simulink model "Pierre_Controller_LPV"  (R2024b)
settings: Solver=ode1  StartTime=0.0  StopTime=inf  FixedStep=Ts  RelTol=1e-3
PostLoadFcn:
  | , if any(exist('dsrtsu_mdlpostloadfcn', 'file') ~= 0), dsrtsu_mdlpostloadfcn('Execute', bdroot); end,
InitFcn:
  | , if any(exist('rtifpga_mdlclblib', 'file') ~= 0), rtifpga_mdlclblib('Init', bdroot); end,
model workspace (MAT data in the model file):
  dmestimate = 1
values from neighbouring files (symbols this model uses):
  BUTTER = ss(A,B,C,D,Ts)    [build_model.m]
  K = opensave.K_final    [build_model.m]
  Px = 1    [build_model.m]
  Py = 1    [build_model.m]
  Pz = 1    [build_model.m]
  S_Sensor = 0.1134    [build_model.m]
  Sen_AX = 2.0176    [build_model.m]
  Sen_AY = 2.011    [build_model.m]
  Sen_AZ = 2.0066    [build_model.m]
  Sen_GX = 0.75481    [build_model.m]
  Sen_GY = 0.75728    [build_model.m]
  Sen_GZ = 0.74931    [build_model.m]
  Sweep_amp = 0.5    [build_model.m]
  Switch_excit = 4    [build_model.m]
  TMS_amp = 2    [build_model.m]
  TMS_freq1 = 80    [build_model.m]
  TMS_freq2 = 0    [build_model.m]
  TMS_freq3 = 0    [build_model.m]
  Ts = 1/Fs    (= 0.001)    [build_model.m]
  V_sat = 2/10    (= 0.2)    [build_model.m]
  V_sat_TMS = 5    [build_model.m]
undefined symbols (not defined in the file or in its folder): dmhat, Gnomden, Gnomnum, R, S
libraries: dspfdesign x15, rti1202lib_adc_class1 x10, rti1202lib_dac_class1 x7, rti1202lib_adc_class2 x6, dspxfrm3 x3, cstblocks x1, simulink x1
(part 3 of 3)

== system Pierre_Controller_LPV/RTI Data ==
  RTI Data Store : Subsystem  Tag="struct('private',struct('version',struct('dsVer',uint32(2),'dsVerCreation',uint32(2),'RTI',struct('ver','7.18','type','RTI1202')),'access',struct('type','Model','isPerm',1,'created',['16-Aug-2022 11:52:04'],'modified',['22-Feb-2023 15:24:02'],'location','')),'public',struct('main',struct('data',[]),'sub',struct('name',{{'Pierre_Controller_LTI'}},'data',{{struct('TH',struct('thTaskInfo',struct('taskType',{'TIMER','HWINT','TMRINT','SWINT','GLINT'},'tasksNumOf',{1,0,0,0,0},'srcIds',{{'TIMERA'},{},{},{},{}},'taskNames',{{['Timer Task 1']},{},{},{},{}})),'th_tc',struct('dataType','TASK','taskGroupId','','taskGroupList',{{}},'taskSchedulingPolicy','FCFS','taskType','TIMER','blkh',-1,'srcId','TIMERA','srcSgnName',['Timer A interrupt'],'srcCpuName','','taskName',['Timer Task 1  [0.001] s'],'taskNameDisplayExt','','smplTime',0.001,'smplTimeOffs',0,'hasFixedPriority',0,'priority',1,'hasFixedOvc',0,'ovcType',1,'ovcMax',1),'tc_th',struct('dataType','TASK','taskGroupId','','taskGroupList',{{}},'taskSchedulingPolicy','FCFS','taskType','TIMER','blkh',-1,'srcId','TIMERA','srcSgnName',['Timer A interrupt'],'srcCpuName','','taskName',['Timer Task 1  [0.001] s'],'taskNameDisplayExt','','smplTime',0.001,'smplTimeOffs',0,'hasFixedPriority',0,'priority',1,'hasFixedOvc',0,'ovcType',1,'ovcMax',1))}})))"  mask(RTI_DATA_STORE){}
      mask help:
      | RTI Data Store Block. This block is used by RTI to store internal model dependent data. Deleting this block will result in data loss.
      |
      | NEVER DELETE, COPY, OR MODIFY THIS BLOCK!
      mask Help:
      | RTI Data Store Block. This block is used by RTI to store internal model dependent data. Deleting this block will result in data loss.
      | 
      | NEVER DELETE, COPY, OR MODIFY THIS BLOCK!
      mask Display: text(0.5, 0.5, ' ', 'HorizontalAlignment', 'center');

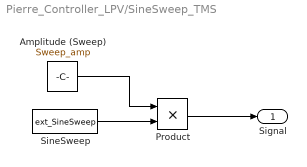
== system Pierre_Controller_LPV/SineSweep_TMS ==
  Amplitude (Sweep) : Constant  Value=Sweep_amp
  Product : Product
  SineSweep : FromWorkspace  VariableName=ext_SineSweep  SampleTime=Ts  Interpolate=off  OutputAfterFinalValue=Cyclic repetition
  Signal : Outport  VectorParamsAs1DForOutWhenUnconnected=off
  wires:
  Product/1 -> Signal/1
  SineSweep/1 -> Product/2
  Amplitude (Sweep)/1 -> Product/1

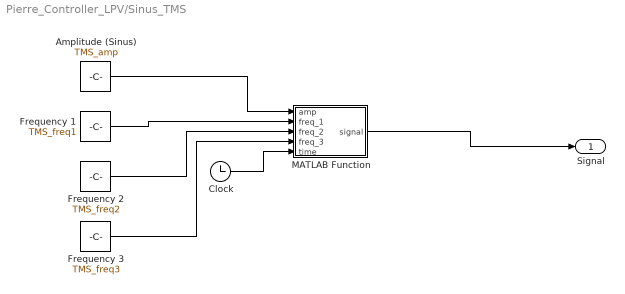
== system Pierre_Controller_LPV/Sinus_TMS ==
  Amplitude (Sinus) : Constant  Value=TMS_amp
  Clock : Clock
  Frequency 1 : Constant  Value=TMS_freq1
  Frequency 2 : Constant  Value=TMS_freq2
  Frequency 3 : Constant  Value=TMS_freq3
  MATLAB Function : MATLAB Function  TreatAsAtomicUnit=on
  Signal : Outport  VectorParamsAs1DForOutWhenUnconnected=off
  wires:
  Frequency 1/1 -> MATLAB Function/2(freq_1)
  Clock/1 -> MATLAB Function/5(time)
  Amplitude (Sinus)/1 -> MATLAB Function/1(amp)
  MATLAB Function/1(signal) -> Signal/1
  Frequency 2/1 -> MATLAB Function/3(freq_2)
  Frequency 3/1 -> MATLAB Function/4(freq_3)

== system Pierre_Controller_LPV/TMS_Command ==
  In1 : Inport
  GainDAC_Ch1 : Gain  Gain=1/10
  Command (V) : Outport  VectorParamsAs1DForOutWhenUnconnected=off
  wires:
  GainDAC_Ch1/1 -> Command (V)/1  "Command (V)"
  In1/1 -> GainDAC_Ch1/1

== system Pierre_Controller_LPV/ARCHIVE/Compensation filter ==
  Reference : Inport
  Compensation filter : cstblocks/LTI System  sys=Cz  IC=[]  PadeOrder=0
  Filtered Reference : Outport  VectorParamsAs1DForOutWhenUnconnected=off
  wires:
  Compensation filter/1 -> Filtered Reference/1
  Reference/1 -> Compensation filter/1

== system Pierre_Controller_LPV/ARCHIVE/SineSweep ==
  Amplitude (Sweep) : Constant
  Product : Product
  SineSweep : FromWorkspace  VariableName=ext_SineSweep  SampleTime=Ts  Interpolate=off  OutputAfterFinalValue=Cyclic repetition
  Signal : Outport  VectorParamsAs1DForOutWhenUnconnected=off
  wires:
  Amplitude (Sweep)/1 -> Product/1
  Product/1 -> Signal/1
  SineSweep/1 -> Product/2

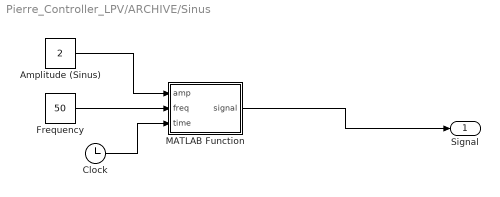
== system Pierre_Controller_LPV/ARCHIVE/Sinus ==
  Amplitude (Sinus) : Constant  Value=2
  Clock : Clock
  Frequency : Constant  Value=50
  MATLAB Function : MATLAB Function  TreatAsAtomicUnit=on
  Signal : Outport  VectorParamsAs1DForOutWhenUnconnected=off
  wires:
  Frequency/1 -> MATLAB Function/2(freq)
  Clock/1 -> MATLAB Function/3(time)
  Amplitude (Sinus)/1 -> MATLAB Function/1(amp)
  MATLAB Function/1(signal) -> Signal/1

== system Pierre_Controller_LPV/Current monitoring/Subsystem ==
  In1 : Inport
  V2A_PMA_monitoring : Gain  Gain=1/5
  PMA1_monitoring (A) : Outport  VectorParamsAs1DForOutWhenUnconnected=off
  wires:
  In1/1 -> V2A_PMA_monitoring/1
  V2A_PMA_monitoring/1 -> PMA1_monitoring (A)/1  "PMA_monitoring (A)"

== system Pierre_Controller_LPV/Current monitoring/Subsystem1 ==
  In1 : Inport
  V2A_PMA_monitoring : Gain  Gain=1/5
  PMA2_monitoring (A) : Outport  VectorParamsAs1DForOutWhenUnconnected=off
  wires:
  In1/1 -> V2A_PMA_monitoring/1
  V2A_PMA_monitoring/1 -> PMA2_monitoring (A)/1  "PMA_monitoring (A)"

== system Pierre_Controller_LPV/Current monitoring/Subsystem2 ==
  In1 : Inport
  V2A_PMA_monitoring : Gain  Gain=1/5
  PMA3_monitoring (A) : Outport  VectorParamsAs1DForOutWhenUnconnected=off
  wires:
  In1/1 -> V2A_PMA_monitoring/1
  V2A_PMA_monitoring/1 -> PMA3_monitoring (A)/1  "PMA_monitoring (A)"

== system Pierre_Controller_LPV/Current monitoring/Subsystem3 ==
  In1 : Inport
  V2A_PMA_monitoring : Gain  Gain=1/5
  PMA4_monitoring (A) : Outport  VectorParamsAs1DForOutWhenUnconnected=off
  wires:
  In1/1 -> V2A_PMA_monitoring/1
  V2A_PMA_monitoring/1 -> PMA4_monitoring (A)/1  "PMA_monitoring (A)"

== system Pierre_Controller_LPV/Current monitoring/Subsystem4 ==
  In1 : Inport
  V2A_PMA_monitoring : Gain  Gain=1/5
  PMA5_monitoring (A) : Outport  VectorParamsAs1DForOutWhenUnconnected=off
  wires:
  In1/1 -> V2A_PMA_monitoring/1
  V2A_PMA_monitoring/1 -> PMA5_monitoring (A)/1  "PMA_monitoring (A)"

== system Pierre_Controller_LPV/Current monitoring/Subsystem5 ==
  In1 : Inport
  V2A_PMA_monitoring : Gain  Gain=1/5
  PMA6_monitoring (A) : Outport  VectorParamsAs1DForOutWhenUnconnected=off
  wires:
  In1/1 -> V2A_PMA_monitoring/1
  V2A_PMA_monitoring/1 -> PMA6_monitoring (A)/1  "PMA_monitoring (A)"

== system Pierre_Controller_LPV/IMU/Subsystem1 ==
  In1 : Inport
  Lowpass Filter : dspfdesign/Lowpass Filter  Commented=through  FilterType=FIR  DesignForMinimumOrder=on  FilterOrder=50  PassbandFrequency=200  StopbandFrequency=400  PassbandRipple=0.1  StopbandAttenuation=80  SampleRateMode=Specify on dialog  SampleRate=Fs  SimulateUsing=Interpreted execution  roundingMode=Floor  coeffsDataTypeStr=fixdt(1,16)
  Gyro_X (rad/s) : Outport  VectorParamsAs1DForOutWhenUnconnected=off
  wires:
  In1/1 -> Lowpass Filter/1
  Lowpass Filter/1 -> Gyro_X (rad/s)/1

== system Pierre_Controller_LPV/IMU/Subsystem12 ==
  In1 : Inport
  Lowpass Filter : dspfdesign/Lowpass Filter  Commented=through  FilterType=FIR  DesignForMinimumOrder=on  FilterOrder=50  PassbandFrequency=200  StopbandFrequency=400  PassbandRipple=0.1  StopbandAttenuation=80  SampleRateMode=Specify on dialog  SampleRate=Fs  SimulateUsing=Interpreted execution  roundingMode=Floor  coeffsDataTypeStr=fixdt(1,16)
  g2ms^2_Wilcoxon : Gain  Gain=9.80655
  Acc_X (m/s^2) : Outport  VectorParamsAs1DForOutWhenUnconnected=off
  wires:
  In1/1 -> g2ms^2_Wilcoxon/1
  g2ms^2_Wilcoxon/1 -> Lowpass Filter/1
  Lowpass Filter/1 -> Acc_X (m/s^2)/1

== system Pierre_Controller_LPV/IMU/Subsystem13 ==
  In1 : Inport
  Lowpass Filter : dspfdesign/Lowpass Filter  Commented=through  FilterType=FIR  DesignForMinimumOrder=on  FilterOrder=50  PassbandFrequency=200  StopbandFrequency=400  PassbandRipple=0.1  StopbandAttenuation=80  SampleRateMode=Specify on dialog  SampleRate=Fs  SimulateUsing=Interpreted execution  roundingMode=Floor  coeffsDataTypeStr=fixdt(1,16)
  g2ms^2_Wilcoxon : Gain  Gain=9.80655
  Acc_Y (m/s^2) : Outport  VectorParamsAs1DForOutWhenUnconnected=off
  wires:
  g2ms^2_Wilcoxon/1 -> Lowpass Filter/1
  In1/1 -> g2ms^2_Wilcoxon/1
  Lowpass Filter/1 -> Acc_Y (m/s^2)/1

== system Pierre_Controller_LPV/IMU/Subsystem14 ==
  In1 : Inport
  Lowpass Filter : dspfdesign/Lowpass Filter  Commented=through  FilterType=FIR  DesignForMinimumOrder=on  FilterOrder=50  PassbandFrequency=200  StopbandFrequency=400  PassbandRipple=0.1  StopbandAttenuation=80  SampleRateMode=Specify on dialog  SampleRate=Fs  SimulateUsing=Interpreted execution  roundingMode=Floor  coeffsDataTypeStr=fixdt(1,16)
  g2ms^2_Wilcoxon : Gain  Gain=9.80655
  Acc_Z (m/s^2) : Outport  VectorParamsAs1DForOutWhenUnconnected=off
  wires:
  In1/1 -> g2ms^2_Wilcoxon/1
  g2ms^2_Wilcoxon/1 -> Lowpass Filter/1
  Lowpass Filter/1 -> Acc_Z (m/s^2)/1

== system Pierre_Controller_LPV/IMU/Subsystem2 ==
  In1 : Inport
  Lowpass Filter : dspfdesign/Lowpass Filter  Commented=through  FilterType=FIR  DesignForMinimumOrder=on  FilterOrder=50  PassbandFrequency=200  StopbandFrequency=400  PassbandRipple=0.1  StopbandAttenuation=80  SampleRateMode=Specify on dialog  SampleRate=Fs  SimulateUsing=Interpreted execution  roundingMode=Floor  coeffsDataTypeStr=fixdt(1,16)
  Gyro_Y (rad/s) : Outport  VectorParamsAs1DForOutWhenUnconnected=off
  wires:
  In1/1 -> Lowpass Filter/1
  Lowpass Filter/1 -> Gyro_Y (rad/s)/1

== system Pierre_Controller_LPV/IMU/Subsystem3 ==
  In1 : Inport
  Lowpass Filter : dspfdesign/Lowpass Filter  Commented=through  FilterType=FIR  DesignForMinimumOrder=on  FilterOrder=50  PassbandFrequency=200  StopbandFrequency=400  PassbandRipple=0.1  StopbandAttenuation=80  SampleRateMode=Specify on dialog  SampleRate=Fs  SimulateUsing=Interpreted execution  roundingMode=Floor  coeffsDataTypeStr=fixdt(1,16)
  Gyro_Z (rad/s) : Outport  VectorParamsAs1DForOutWhenUnconnected=off
  wires:
  In1/1 -> Lowpass Filter/1
  Lowpass Filter/1 -> Gyro_Z (rad/s)/1

== system Pierre_Controller_LPV/PMA Accelerometers/Subsystem10 ==
  In1 : Inport
  Lowpass Filter : dspfdesign/Lowpass Filter  Commented=through  FilterType=FIR  DesignForMinimumOrder=on  FilterOrder=50  PassbandFrequency=300  StopbandFrequency=500  PassbandRipple=0.1  StopbandAttenuation=80  SampleRateMode=Specify on dialog  SampleRate=Fs  SimulateUsing=Interpreted execution  roundingMode=Floor  coeffsDataTypeStr=fixdt(1,16)
  g2ms^2_Micromega : Gain  Gain=9.8105
  g2ms^2_Micromega5 : Outport  VectorParamsAs1DForOutWhenUnconnected=off
  wires:
  In1/1 -> g2ms^2_Micromega/1
  g2ms^2_Micromega/1 -> Lowpass Filter/1
  Lowpass Filter/1 -> g2ms^2_Micromega5/1

== system Pierre_Controller_LPV/PMA Accelerometers/Subsystem11 ==
  In1 : Inport
  Lowpass Filter : dspfdesign/Lowpass Filter  Commented=through  FilterType=FIR  DesignForMinimumOrder=on  FilterOrder=50  PassbandFrequency=300  StopbandFrequency=500  PassbandRipple=0.1  StopbandAttenuation=80  SampleRateMode=Specify on dialog  SampleRate=Fs  SimulateUsing=Interpreted execution  roundingMode=Floor  coeffsDataTypeStr=fixdt(1,16)
  g2ms^2_Micromega : Gain  Gain=9.8105
  g2ms^2_Micromega6 : Outport  VectorParamsAs1DForOutWhenUnconnected=off
  wires:
  g2ms^2_Micromega/1 -> Lowpass Filter/1
  In1/1 -> g2ms^2_Micromega/1
  Lowpass Filter/1 -> g2ms^2_Micromega6/1

== system Pierre_Controller_LPV/PMA Accelerometers/Subsystem6 ==
  In1 : Inport
  Lowpass Filter : dspfdesign/Lowpass Filter  Commented=through  FilterType=FIR  DesignForMinimumOrder=on  FilterOrder=50  PassbandFrequency=300  StopbandFrequency=500  PassbandRipple=0.1  StopbandAttenuation=80  SampleRateMode=Specify on dialog  SampleRate=Fs  SimulateUsing=Interpreted execution  roundingMode=Floor  coeffsDataTypeStr=fixdt(1,16)
  g2ms^2_Micromega : Gain  Gain=9.8105
  g2ms^2_Micromega1 : Outport  VectorParamsAs1DForOutWhenUnconnected=off
  wires:
  g2ms^2_Micromega/1 -> Lowpass Filter/1
  In1/1 -> g2ms^2_Micromega/1
  Lowpass Filter/1 -> g2ms^2_Micromega1/1

== system Pierre_Controller_LPV/PMA Accelerometers/Subsystem7 ==
  In1 : Inport
  Lowpass Filter : dspfdesign/Lowpass Filter  Commented=through  FilterType=FIR  DesignForMinimumOrder=on  FilterOrder=50  PassbandFrequency=300  StopbandFrequency=500  PassbandRipple=0.1  StopbandAttenuation=80  SampleRateMode=Specify on dialog  SampleRate=Fs  SimulateUsing=Interpreted execution  roundingMode=Floor  coeffsDataTypeStr=fixdt(1,16)
  g2ms^2_Micromega : Gain  Gain=9.8105
  g2ms^2_Micromega2 : Outport  VectorParamsAs1DForOutWhenUnconnected=off
  wires:
  g2ms^2_Micromega/1 -> Lowpass Filter/1
  In1/1 -> g2ms^2_Micromega/1
  Lowpass Filter/1 -> g2ms^2_Micromega2/1

== system Pierre_Controller_LPV/PMA Accelerometers/Subsystem8 ==
  In1 : Inport
  Lowpass Filter : dspfdesign/Lowpass Filter  Commented=through  FilterType=FIR  DesignForMinimumOrder=on  FilterOrder=50  PassbandFrequency=300  StopbandFrequency=500  PassbandRipple=0.1  StopbandAttenuation=80  SampleRateMode=Specify on dialog  SampleRate=Fs  SimulateUsing=Interpreted execution  roundingMode=Floor  coeffsDataTypeStr=fixdt(1,16)
  g2ms^2_Micromega : Gain  Gain=9.8105
  g2ms^2_Micromega3 : Outport  VectorParamsAs1DForOutWhenUnconnected=off
  wires:
  g2ms^2_Micromega/1 -> Lowpass Filter/1
  In1/1 -> g2ms^2_Micromega/1
  Lowpass Filter/1 -> g2ms^2_Micromega3/1

== system Pierre_Controller_LPV/PMA Accelerometers/Subsystem9 ==
  In1 : Inport
  Lowpass Filter : dspfdesign/Lowpass Filter  Commented=through  FilterType=FIR  DesignForMinimumOrder=on  FilterOrder=50  PassbandFrequency=300  StopbandFrequency=500  PassbandRipple=0.1  StopbandAttenuation=80  SampleRateMode=Specify on dialog  SampleRate=Fs  SimulateUsing=Interpreted execution  roundingMode=Floor  coeffsDataTypeStr=fixdt(1,16)
  g2ms^2_Micromega : Gain  Gain=9.8105
  g2ms^2_Micromega4 : Outport  VectorParamsAs1DForOutWhenUnconnected=off
  wires:
  g2ms^2_Micromega/1 -> Lowpass Filter/1
  In1/1 -> g2ms^2_Micromega/1
  Lowpass Filter/1 -> g2ms^2_Micromega4/1

== system Pierre_Controller_LPV/Payload Accelerometers/Subsystem12 ==
  In1 : Inport
  Lowpass Filter : dspfdesign/Lowpass Filter  Commented=through  FilterType=FIR  DesignForMinimumOrder=on  FilterOrder=50  PassbandFrequency=200  StopbandFrequency=400  PassbandRipple=0.1  StopbandAttenuation=80  SampleRateMode=Specify on dialog  SampleRate=Fs  SimulateUsing=Interpreted execution  roundingMode=Floor  coeffsDataTypeStr=fixdt(1,16)
  g2ms^2_Wilcoxon : Gain  Gain=9.80655
  g2ms^2_Wilcoxon1 : Outport  VectorParamsAs1DForOutWhenUnconnected=off
  wires:
  In1/1 -> g2ms^2_Wilcoxon/1
  g2ms^2_Wilcoxon/1 -> Lowpass Filter/1
  Lowpass Filter/1 -> g2ms^2_Wilcoxon1/1

== system Pierre_Controller_LPV/Payload Accelerometers/Subsystem13 ==
  In1 : Inport
  Lowpass Filter : dspfdesign/Lowpass Filter  Commented=through  FilterType=FIR  DesignForMinimumOrder=on  FilterOrder=50  PassbandFrequency=200  StopbandFrequency=400  PassbandRipple=0.1  StopbandAttenuation=80  SampleRateMode=Specify on dialog  SampleRate=Fs  SimulateUsing=Interpreted execution  roundingMode=Floor  coeffsDataTypeStr=fixdt(1,16)
  g2ms^2_Wilcoxon : Gain  Gain=9.80655
  g2ms^2_Wilcoxon2 : Outport  VectorParamsAs1DForOutWhenUnconnected=off
  wires:
  g2ms^2_Wilcoxon/1 -> Lowpass Filter/1
  In1/1 -> g2ms^2_Wilcoxon/1
  Lowpass Filter/1 -> g2ms^2_Wilcoxon2/1

== system Pierre_Controller_LPV/Payload Accelerometers/Subsystem14 ==
  In1 : Inport
  Lowpass Filter : dspfdesign/Lowpass Filter  Commented=through  FilterType=FIR  DesignForMinimumOrder=on  FilterOrder=50  PassbandFrequency=200  StopbandFrequency=400  PassbandRipple=0.1  StopbandAttenuation=80  SampleRateMode=Specify on dialog  SampleRate=Fs  SimulateUsing=Interpreted execution  roundingMode=Floor  coeffsDataTypeStr=fixdt(1,16)
  g2ms^2_Wilcoxon : Gain  Gain=9.80655
  g2ms^2_Wilcoxon3 : Outport  VectorParamsAs1DForOutWhenUnconnected=off
  wires:
  In1/1 -> g2ms^2_Wilcoxon/1
  g2ms^2_Wilcoxon/1 -> Lowpass Filter/1
  Lowpass Filter/1 -> g2ms^2_Wilcoxon3/1

== system Pierre_Controller_LPV/RTI Data/RTI Data Store ==
  RTI Data Store : Subsystem  mask(RTI_DATA_STORE){}
      mask help:
      | RTI Data Store Block. This block is used by RTI to store internal model dependent data. Deleting this block will result in data loss.
      |
      | NEVER DELETE, COPY, OR MODIFY THIS BLOCK!
      mask Help:
      | RTI Data Store Block. This block is used by RTI to store internal model dependent data. Deleting this block will result in data loss.
      | 
      | NEVER DELETE, COPY, OR MODIFY THIS BLOCK!
      mask Display: text(0.5, 0.5, ' ', 'HorizontalAlignment', 'center');

== system Pierre_Controller_LPV/RTI Data/RTI Data Store/RTI Data Store ==
  RTI Data Store : Subsystem  mask(RTI_DATA_STORE){}
      mask help:
      | RTI Data Store Block. This block is used by RTI to store internal model dependent data. Deleting this block will result in data loss.
      |
      | NEVER DELETE, COPY, OR MODIFY THIS BLOCK!
      mask Help:
      | RTI Data Store Block. This block is used by RTI to store internal model dependent data. Deleting this block will result in data loss.
      | 
      | NEVER DELETE, COPY, OR MODIFY THIS BLOCK!
      mask Display: text(0.5, 0.5, ' ', 'HorizontalAlignment', 'center');

== system Pierre_Controller_LPV/RTI Data/RTI Data Store/RTI Data Store/RTI Data Store ==
  RTI Data Store : Subsystem  mask(RTI_DATA_STORE){}
      mask help:
      | RTI Data Store Block. This block is used by RTI to store internal model dependent data. Deleting this block will result in data loss.
      |
      | NEVER DELETE, COPY, OR MODIFY THIS BLOCK!
      mask Help:
      | RTI Data Store Block. This block is used by RTI to store internal model dependent data. Deleting this block will result in data loss.
      | 
      | NEVER DELETE, COPY, OR MODIFY THIS BLOCK!
      mask Display: text(0.5, 0.5, ' ', 'HorizontalAlignment', 'center');

== system Pierre_Controller_LPV/RTI Data/RTI Data Store/RTI Data Store/RTI Data Store/RTI Data Store ==

== matlab function Pierre_Controller_LPV/MATLAB Function ==
  data: exc input; u_exc_cmd output; Exc_Route input; u_exc_dist output
function [u_exc_cmd, u_exc_dist] = Exc_Router(exc, Exc_Route)
% Exc_Route: 0 = disturbance (shaker), 1 = command (PMA)
if Exc_Route == 1
    u_exc_cmd  = exc;
    u_exc_dist = 0;
else
    u_exc_cmd  = 0;
    u_exc_dist = exc;
end

== matlab function Pierre_Controller_LPV/Harmonics Estimator/SDFT ==
  data: DFT_out output; x input; init input; iter_out output
function [DFT_out, iter_out]  = SDFT(x, init)
% Compute DFT of x recursively with sliding window
% N corresponds to the number of samplings to accumulate for first FFT
% computation (during 1 second)

persistent signal iter DFT % N

% Initialize parameters
if isempty(signal)
    %N = 1/Ts;
    iter = 0;
    signal = zeros(1,1000);
    DFT = complex(zeros(1,1000));
end

%N = 1/Ts;

if isequal(init,1)
    signal = zeros(1,1000);
end
iter = iter+1;
iter_out = iter;

% Accumulate N samples to initialize algorithm
if iter < 1001
    signal(iter) = x;
%     signal_out = zeros(1,1000);
    vec = 0:iter-1;
    DFT(iter) = DFT(iter-1)+(signal(vec)*exp(-1j*2*pi*vec/1000));
    DFT_out = DFT;

%     for k = 1:iter
% %         k = 1;
%         DFT(k) = 0;
%         for n = 1:iter
% %             n = 1;   
%             DFT(k) = DFT(k) + (signal(n)*exp((-1j)*2*pi*(n-1)*(k-1)/1000));
%         end
%     end
    
%     peak_freq = zeros(1,5);

% Compute DFT after first N samples
% elseif isequal(iter,1000)
%     signal(iter) = x;
% %     DFT_out = complex(zeros(1,1000));
% %     DFT = DFT_out;
%     signal_out = signal;
% 
%     vec = 0:1000-1;
%     DFT(iter) = DFT(iter-1)+(signal(n)*exp(-1j*2*pi*vec/1000));
%     

%     peak_freq = getPeaks(DFT,Ts,1000);
    

% Recursive update of DFT
else
%     oldest_value = signal(1);
%     if isequal(iter, 1001)
%         DFT = DFT_in;
%     end
    vec = 0:1000-1;
    DFT = (DFT-signal(1)+x).*exp(1j*2*pi*vec/1000);
    DFT_out = DFT;
%     DFT = fft(signal);
%     DFT = complex(zeros(1,1000));

    signal = [signal(2:end) x];
%     signal_out = signal;
%     peak_freq = getPeaks(DFT,Ts,1000);
end

end

% function peak_freq = getPeaks(DFT,Ts,N)
% N_2 = ceil(1000/2);
% freq = 0:1:N_2-1;
% peak_freq = zeros(1,5);
% [~,index] = findpeaks(abs(DFT(1:N_2)),'MinPeakHeight', 10);
% for n = 1:length(index)
%     if isequal(n,6)
%         break
%     end
%     peak_freq(n) = freq(index(n));  %[Hz]
% end
% end

== matlab function Pierre_Controller_LPV/Sinus_TMS/MATLAB Function ==
  data: amp input; freq_1 input; freq_2 input; freq_3 input; signal output; time input
function signal = Sinus(amp,freq_1,freq_2,freq_3,time)

signal = amp*(sin(2*pi*freq_1*time)+sin(2*pi*freq_2*time)+sin(2*pi*freq_3*time));

end

== matlab function Pierre_Controller_LPV/Harmonics Estimator/SDFT_x ==
  data: x input; Ts input; peak_freq output size=[1,5]; init input; iter_out output
function [peak_freq, iter_out] = SDFT(x, Ts, init)
% Compute DFT of x recursively with sliding window
% N corresponds to the number of samplings to accumulate for first FFT
% computation (during 1 second)

persistent signal DFT iter % N

% Initialize parameters
if isempty(signal)
    %N = 1/Ts;
    iter = 0;
    signal = zeros(1,1000);
    DFT = zeros(1,1000);
end

%N = 1/Ts;

if isequal(init,1)
    signal = zeros(1,1000);
end
iter = iter+1;
iter_out = iter;

% Accumulate N samples to initialize algorithm
if iter < 1000
    signal(iter) = x;
    peak_freq = zeros(1,5);

% Compute DFT after first N samples
elseif isequal(iter,1000)
    signal(iter) = x;
%     DFT = fft(signal);
    temp = zeros(1,1000);
    DFT = complex(temp);
    for k = 1:1000
        DFT(k) = 0;
        for n = 1:1000
            DFT(k) = DFT(k)+(signal(n)*exp((-1j)*2*pi*(n-1)*(k-1)/1000));
        end
    end
    peak_freq = getPeaks(DFT,Ts,1000);

% Recursive update of DFT
else
    oldest_value = signal(1);
    DFT = (DFT-signal(1)+x).*exp(j*2*pi*[0:1000-1]/1000);
    signal = [signal(2:end) x];
    peak_freq = getPeaks(DFT,Ts,1000);
end

end

function peak_freq = getPeaks(DFT,Ts,N)
N_2 = ceil(1000/2);
freq = 0:1:N_2-1;
peak_freq = zeros(1,5);
[~,index] = findpeaks(abs(DFT(1:N_2)),'MinPeakHeight', 10);
for n = 1:length(index)
    if isequal(n,6)
        break
    end
    peak_freq(n) = freq(index(n));  %[Hz]
end
end

== matlab function Pierre_Controller_LPV/Harmonics Estimator/SDFT_y ==
  data: x input; Ts input; peak_freq output size=[1,5]; init input
function peak_freq = SDFT(x, Ts, init)
% Compute DFT of x recursively with sliding window
% N corresponds to the number of samplings to accumulate for first FFT
% computation (during 1 second)

persistent signal DFT iter % N

% Initialize parameters
if isempty(signal)
%     N = 1/Ts;
    iter = 0;
    signal = zeros(1,1000);
    DFT = zeros(1,1000);
end

if isequal(init,1)
    signal = zeros(1,1000);
end
iter = iter+1;

% Accumulate N samples to initialize algorithm
if iter < 1000
    signal(iter) = x;
    peak_freq = zeros(1,5);

% Compute DFT after first N samples
elseif isequal(iter,1000)
    signal(iter) = x;
    DFT = fft(signal);
    peak_freq = getPeaks(DFT,Ts,1000);

% Recursive update of DFT
else
    oldest_value = signal(1);
    DFT = (DFT-signal(1)+x).*exp(j*2*pi*[0:1000-1]/1000);
    signal = [signal(2:end) x];
    peak_freq = getPeaks(DFT,Ts,1000);
end

end

function peak_freq = getPeaks(DFT,Ts,N)
N_2 = ceil(1000/2);
freq = 0:1:N_2-1;
peak_freq = zeros(1,5);
[~,index] = findpeaks(abs(DFT(1:N_2)),'MinPeakHeight', 10);
for n = 1:length(index)
    if isequal(n,6)
        break
    end
    peak_freq(n) = freq(index(n));  %[Hz]
end
end

== matlab function Pierre_Controller_LPV/Harmonics Estimator/SDFT_z ==
  data: x input; Ts input; peak_freq output size=[1,5]; init input
function peak_freq = SDFT(x, Ts, init)
% Compute DFT of x recursively with sliding window
% N corresponds to the number of samplings to accumulate for first FFT
% computation (during 1 second)

persistent signal DFT iter % N

% Initialize parameters
if isempty(signal)
%     N = 1/Ts;
    iter = 0;
    signal = zeros(1,1000);
    DFT = zeros(1,1000);
end

if isequal(init,1)
    signal = zeros(1,1000);
end
iter = iter+1;

% Accumulate N samples to initialize algorithm
if iter < 1000
    signal(iter) = x;
    peak_freq = zeros(1,5);

% Compute DFT after first N samples
elseif isequal(iter,1000)
    signal(iter) = x;
    DFT = fft(signal);
    peak_freq = getPeaks(DFT,Ts,1000);

% Recursive update of DFT
else
    oldest_value = signal(1);
    DFT = (DFT-signal(1)+x).*exp(j*2*pi*[0:1000-1]/1000);
    signal = [signal(2:end) x];
    peak_freq = getPeaks(DFT,Ts,1000);
end

end

function peak_freq = getPeaks(DFT,Ts,N)
N_2 = ceil(1000/2);
freq = 0:1:N_2-1;
peak_freq = zeros(1,5);
[~,index] = findpeaks(abs(DFT(1:N_2)),'MinPeakHeight', 10);
for n = 1:length(index)
    if isequal(n,6)
        break
    end
    peak_freq(n) = freq(index(n));  %[Hz]
end
end

== matlab function Pierre_Controller_LPV/Harmonics Estimator/MATLAB Function8 ==
  data: DFT input; Ts input; peak_freq output size=[1,3]
function peak_freq = getPeaks(DFT,Ts)
N_2 = ceil(1/2/Ts);
freq = zeros(1,500);
freq = 0:1:500-1;
peak_freq = zeros(1,3);
[~,index] = findpeaks(abs(DFT(1:N_2)),'MinPeakHeight', 0.05);
for n = 1:length(index)
    if isequal(n,4)
        break
    end
    if freq(index(n)) > 29
        peak_freq(n) = freq(index(n));  %[Hz]
    else peak_freq(n) = 0;
    end
end
